simulink model "Simu1Motor"  (R2025b)
settings: Solver=VariableStepAuto  StartTime=0.0  StopTime=10  RelTol=1e-3
undefined symbols (not defined in the file): aa1, alpha, bb3, bc, c0, c1, den, dspblkCoreblockFVToolHelper, gcbh, gfz, GT_num, HT_num, K, Ka, ki, Ko, Kos, kp, num, r1, ra, s0, s1, Tm, Tm1
libraries: simulink x1
settings Model: Creator=Administrador  LastModifiedBy=User

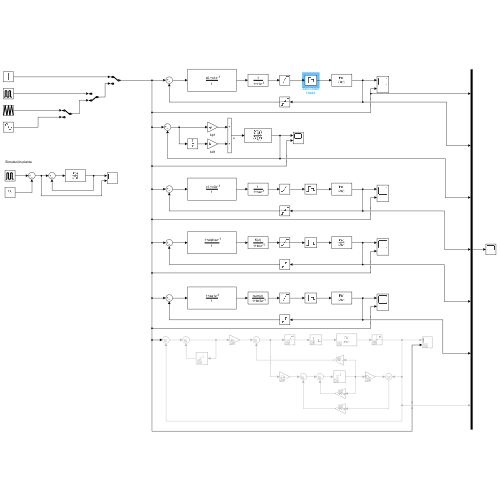
[thumbnail: Simulink's stored preview of the top-level diagram]
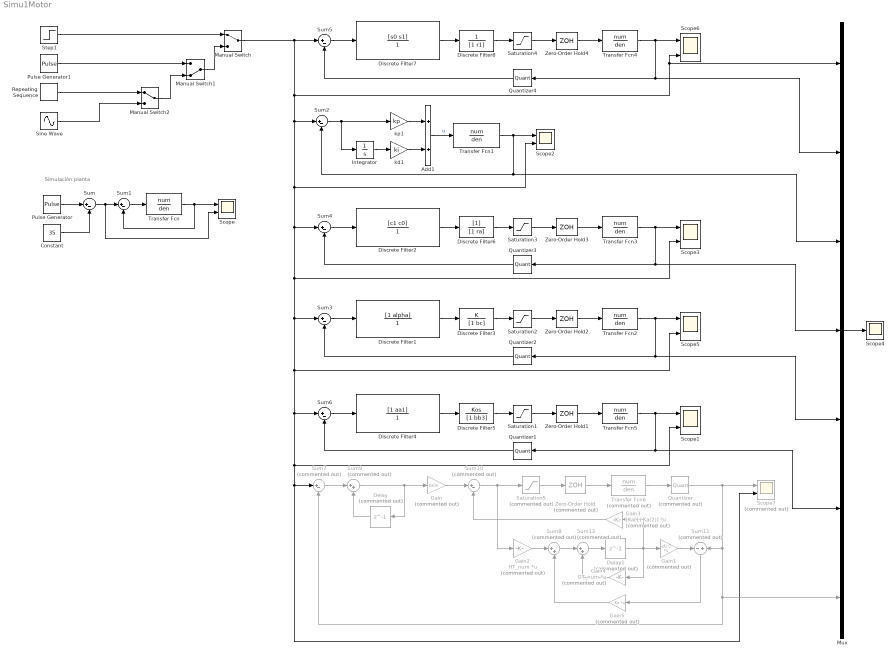
== system Simu1Motor ==
  note: Simulación planta
  Add1 : Sum
  Constant : Constant  Value=35
  Delay : Delay  Commented=on  DelayLength=1  InputProcessing=Columns as channels (frame based)  SampleTime=Tm
  Delay1 : Delay  Commented=on  DelayLength=1  InputProcessing=Columns as channels (frame based)  SampleTime=Tm
  Discrete Filter1 : DiscreteFilter  LoadFcn=dspblkCoreblockFVToolHelper(gcbh,'load');  Numerator=[1 alpha]  Denominator=1
      settings: CopyFcn=dspblkCoreblockFVToolHelper(gcbh,'copy');  DeleteFcn=dspblkCoreblockFVToolHelper(gcbh,'close');  ModelCloseFcn=dspblkCoreblockFVToolHelper(gcbh,'close');  PreSaveFcn=dspblkCoreblockFVToolHelper(gcbh,'presave');  PostSaveFcn=dspblkCoreblockFVToolHelper(gcbh,'postsave');  CloseFcn=dspblkCoreblockFVToolHelper(gcbh,'close');
  Discrete Filter2 : DiscreteFilter  LoadFcn=dspblkCoreblockFVToolHelper(gcbh,'load');  Numerator=[c1 c0]  Denominator=1
      settings: CopyFcn=dspblkCoreblockFVToolHelper(gcbh,'copy');  DeleteFcn=dspblkCoreblockFVToolHelper(gcbh,'close');  ModelCloseFcn=dspblkCoreblockFVToolHelper(gcbh,'close');  PreSaveFcn=dspblkCoreblockFVToolHelper(gcbh,'presave');  PostSaveFcn=dspblkCoreblockFVToolHelper(gcbh,'postsave');  CloseFcn=dspblkCoreblockFVToolHelper(gcbh,'close');
  Discrete Filter3 : DiscreteFilter  LoadFcn=dspblkCoreblockFVToolHelper(gcbh,'load');  Numerator=K  Denominator=[1 bc]
      settings: CopyFcn=dspblkCoreblockFVToolHelper(gcbh,'copy');  DeleteFcn=dspblkCoreblockFVToolHelper(gcbh,'close');  ModelCloseFcn=dspblkCoreblockFVToolHelper(gcbh,'close');  PreSaveFcn=dspblkCoreblockFVToolHelper(gcbh,'presave');  PostSaveFcn=dspblkCoreblockFVToolHelper(gcbh,'postsave');  CloseFcn=dspblkCoreblockFVToolHelper(gcbh,'close');
  Discrete Filter4 : DiscreteFilter  LoadFcn=dspblkCoreblockFVToolHelper(gcbh,'load');  Numerator=[1 aa1]  Denominator=1
      settings: CopyFcn=dspblkCoreblockFVToolHelper(gcbh,'copy');  DeleteFcn=dspblkCoreblockFVToolHelper(gcbh,'close');  ModelCloseFcn=dspblkCoreblockFVToolHelper(gcbh,'close');  PreSaveFcn=dspblkCoreblockFVToolHelper(gcbh,'presave');  PostSaveFcn=dspblkCoreblockFVToolHelper(gcbh,'postsave');  CloseFcn=dspblkCoreblockFVToolHelper(gcbh,'close');
  Discrete Filter5 : DiscreteFilter  LoadFcn=dspblkCoreblockFVToolHelper(gcbh,'load');  Numerator=Kos  Denominator=[1 bb3]
      settings: CopyFcn=dspblkCoreblockFVToolHelper(gcbh,'copy');  DeleteFcn=dspblkCoreblockFVToolHelper(gcbh,'close');  ModelCloseFcn=dspblkCoreblockFVToolHelper(gcbh,'close');  PreSaveFcn=dspblkCoreblockFVToolHelper(gcbh,'presave');  PostSaveFcn=dspblkCoreblockFVToolHelper(gcbh,'postsave');  CloseFcn=dspblkCoreblockFVToolHelper(gcbh,'close');
  Discrete Filter6 : DiscreteFilter  LoadFcn=dspblkCoreblockFVToolHelper(gcbh,'load');  Denominator=[1 ra]
      settings: CopyFcn=dspblkCoreblockFVToolHelper(gcbh,'copy');  DeleteFcn=dspblkCoreblockFVToolHelper(gcbh,'close');  ModelCloseFcn=dspblkCoreblockFVToolHelper(gcbh,'close');  PreSaveFcn=dspblkCoreblockFVToolHelper(gcbh,'presave');  PostSaveFcn=dspblkCoreblockFVToolHelper(gcbh,'postsave');  CloseFcn=dspblkCoreblockFVToolHelper(gcbh,'close');
  Discrete Filter7 : DiscreteFilter  LoadFcn=dspblkCoreblockFVToolHelper(gcbh,'load');  Numerator=[s0 s1]  Denominator=1
      settings: CopyFcn=dspblkCoreblockFVToolHelper(gcbh,'copy');  DeleteFcn=dspblkCoreblockFVToolHelper(gcbh,'close');  ModelCloseFcn=dspblkCoreblockFVToolHelper(gcbh,'close');  PreSaveFcn=dspblkCoreblockFVToolHelper(gcbh,'presave');  PostSaveFcn=dspblkCoreblockFVToolHelper(gcbh,'postsave');  CloseFcn=dspblkCoreblockFVToolHelper(gcbh,'close');
  Discrete Filter8 : DiscreteFilter  LoadFcn=dspblkCoreblockFVToolHelper(gcbh,'load');  Numerator=1  Denominator=[1 r1]
      settings: CopyFcn=dspblkCoreblockFVToolHelper(gcbh,'copy');  DeleteFcn=dspblkCoreblockFVToolHelper(gcbh,'close');  ModelCloseFcn=dspblkCoreblockFVToolHelper(gcbh,'close');  PreSaveFcn=dspblkCoreblockFVToolHelper(gcbh,'presave');  PostSaveFcn=dspblkCoreblockFVToolHelper(gcbh,'postsave');  CloseFcn=dspblkCoreblockFVToolHelper(gcbh,'close');
  Gain : Gain  Commented=on  Gain=Ka(3)
  Gain1 : Gain  Commented=on  Gain=gfz.C  Multiplication=Matrix(K*u)
  Gain2 : Gain  Commented=on  Gain=HT_num  Multiplication=Matrix(K*u)
  Gain3 : Gain  Commented=on  Gain=[Ka(1) Ka(2)]  Multiplication=Matrix(K*u)
  Gain4 : Gain  Commented=on  Gain=GT_num  Multiplication=Matrix(K*u)
  Gain5 : Gain  Commented=on  Gain=Ko  Multiplication=Matrix(K*u)
  Integrator : Integrator
  Manual Switch : ManualSwitch
  Manual Switch1 : ManualSwitch  CurrentSetting=0
  Manual Switch2 : ManualSwitch
  Mux : Mux  Inputs=7
  Pulse Generator : DiscretePulseGenerator  PulseType=Time based  Amplitude=70  Period=0.8  PulseWidth=50
  Pulse Generator1 : DiscretePulseGenerator  PulseType=Time based  Period=0.8  PulseWidth=50
  Quantizer : Quantizer  Commented=on  QuantizationInterval=5/(2^10)
  Quantizer{1..4} (4 alike) : Quantizer  QuantizationInterval=5/(2^10)
  Repeating Sequence : simulink/Sources/Repeating Sequence  rep_seq_t=[0 1 2]  rep_seq_y=[0 1 0]
  Saturation{1..4} (4 alike) : Saturate  UpperLimit=60  LowerLimit=-60
  Saturation5 : Saturate  Commented=on  UpperLimit=60  LowerLimit=-60
  Scope{,1..3,5..6} (6 alike) : Scope  NumInputPorts=2
      Scope settings: ActiveDisplayYMinimum=-43.75  ActiveDisplayYMaximum=43.75
      Scope1 settings: ActiveDisplayYMinimum=-0.12524414228055636  ActiveDisplayYMaximum=1.1271972805250075
      Scope2 settings: ActiveDisplayYMinimum=-0.125  ActiveDisplayYMaximum=1.125  DataLoggingVariableName=ScopeData4
      Scope3 settings: ActiveDisplayYMinimum=-0.125  ActiveDisplayYMaximum=1.125  DataLoggingVariableName=ScopeData5
      Scope5 settings: ActiveDisplayYMinimum=-0.16141581808620467  ActiveDisplayYMaximum=1.4527423627758422  DataLoggingVariableName=ScopeData6
      Scope6 settings: ActiveDisplayYMinimum=-1.24999  ActiveDisplayYMaximum=1.24999
  Scope4 : Scope
      settings: ActiveDisplayYMinimum=-0.14020975655024898  ActiveDisplayYMaximum=1.261887808952241
  Scope7 : Scope  Commented=on  NumInputPorts=2
      settings: ActiveDisplayYMinimum=-41.17859  ActiveDisplayYMaximum=56.10535
  Sine Wave : Sin  Frequency=5  SampleTime=0
  Step1 : Step  SampleTime=0
  Sum{,1..6} (7 alike) : Sum  Inputs=|+-
  Sum10 : Sum  Commented=on  Inputs=|+-
  Sum11 : Sum  Commented=on  Inputs=-+
  Sum12 : Sum  Commented=on  Inputs=|++
  Sum7 : Sum  Commented=on  Inputs=|+-
  Sum8 : Sum  Commented=on  Inputs=|++
  Sum9 : Sum  Commented=on  Inputs=|++
  Transfer Fcn{,1..5} (6 alike) : TransferFcn  Numerator=num  Denominator=den
  Transfer Fcn6 : TransferFcn  Commented=on  Numerator=num  Denominator=den
  Zero-Order Hold : ZeroOrderHold  Commented=on  SampleTime=Tm
  Zero-Order Hold1 : ZeroOrderHold  SampleTime=Tm1
  Zero-Order Hold2 : ZeroOrderHold  SampleTime=Tm
  Zero-Order Hold3 : ZeroOrderHold  SampleTime=Tm
  Zero-Order Hold4 : ZeroOrderHold  SampleTime=Tm
  kd1 : Gain  Gain=ki
  kp1 : Gain  Gain=kp
  wires:
  Transfer Fcn/1 -> Sum1/2, Scope/1
  Sum1/1 -> Transfer Fcn/1
  Sum/1 -> Scope/2, Sum1/1
  Pulse Generator/1 -> Sum/1
  Constant/1 -> Sum/2
  Pulse Generator1/1 -> Manual Switch1/1
  Step1/1 -> Manual Switch/1
  Manual Switch1/1 -> Manual Switch/2
  Repeating Sequence/1 -> Manual Switch2/1
  Manual Switch2/1 -> Manual Switch1/2
  Sine Wave/1 -> Manual Switch2/2
  kd1/1 -> Add1/2
  Integrator/1 -> kd1/1
  Transfer Fcn1/1 -> Scope2/1, Mux/3, Sum2/2
  kp1/1 -> Add1/1
  Sum2/1 -> Integrator/1, kp1/1
  Add1/1 -> Transfer Fcn1/1  "u"
  Discrete Filter2/1 -> Discrete Filter6/1
  Discrete Filter6/1 -> Saturation3/1
  Saturation3/1 -> Zero-Order Hold3/1
  Transfer Fcn3/1 -> Quantizer3/1, Mux/4, Scope3/1
  Quantizer3/1 -> Sum4/2
  Zero-Order Hold3/1 -> Transfer Fcn3/1
  Sum4/1 -> Discrete Filter2/1
  Mux/1 -> Scope4/1
  Sum3/1 -> Discrete Filter1/1
  Saturation2/1 -> Zero-Order Hold2/1
  Quantizer2/1 -> Sum3/2
  Transfer Fcn2/1 -> Quantizer2/1, Mux/5, Scope5/1
  Zero-Order Hold2/1 -> Transfer Fcn2/1
  Discrete Filter3/1 -> Saturation2/1
  Discrete Filter1/1 -> Discrete Filter3/1
  Saturation4/1 -> Zero-Order Hold4/1
  Quantizer4/1 -> Sum5/2
  Sum5/1 -> Discrete Filter7/1
  Discrete Filter7/1 -> Discrete Filter8/1
  Transfer Fcn4/1 -> Mux/2, Quantizer4/1, Scope6/1
  Zero-Order Hold4/1 -> Transfer Fcn4/1
  Discrete Filter8/1 -> Saturation4/1
  Zero-Order Hold1/1 -> Transfer Fcn5/1
  Quantizer1/1 -> Sum6/2
  Discrete Filter4/1 -> Discrete Filter5/1
  Transfer Fcn5/1 -> Quantizer1/1, Mux/6, Scope1/1
  Sum6/1 -> Discrete Filter4/1
  Saturation1/1 -> Zero-Order Hold1/1
  Discrete Filter5/1 -> Saturation1/1
  Zero-Order Hold/1 -> Transfer Fcn6/1
  Gain/1 -> Sum10/1
  Gain1/1 -> Sum11/1
  Sum9/1 -> Delay/1, Gain/1
  Transfer Fcn6/1 -> Quantizer/1
  Delay1/1 -> Gain3/1, Gain4/1, Gain1/1
  Sum10/1 -> Gain2/1, Saturation5/1
  Sum8/1 -> Sum12/1
  Manual Switch/1 -> Scope6/2, Mux/1, Scope7/2, Sum7/1, Scope1/2, Sum6/1, Scope5/2, Sum3/1, Scope3/2, Sum4/1, Scope2/2, Sum2/1, Sum5/1
  Gain2/1 -> Sum8/1
  Sum7/1 -> Sum9/1
  Saturation5/1 -> Zero-Order Hold/1
  Delay/1 -> Sum9/2
  Sum12/1 -> Delay1/1
  Gain5/1 -> Sum8/2
  Sum11/1 -> Gain5/1
  Gain4/1 -> Sum12/2
  Quantizer/1 -> Mux/7, Sum7/2, Sum11/2, Scope7/1
  Gain3/1 -> Sum10/2
